simulink model "Es4_simulink"  (R2025b)
settings: Solver=VariableStepAuto  StartTime=0.0  StopTime=10.0  RelTol=1e-3
undefined symbols (not defined in the file): const_expr1, const_expr2, ramp_gain, step_gain
libraries: simulink x1
settings Model: Creator=fsisa  LastModifiedBy=fsisa

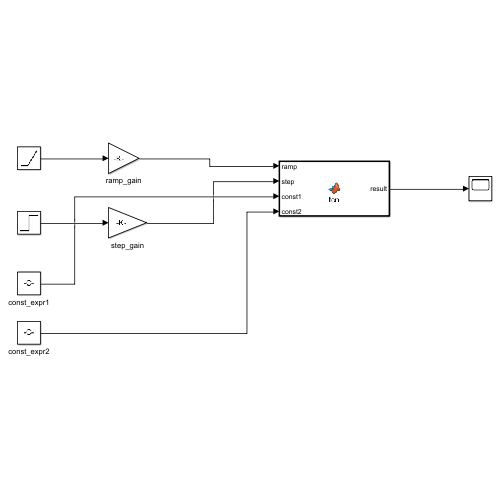
[thumbnail: Simulink's stored preview of the top-level diagram]
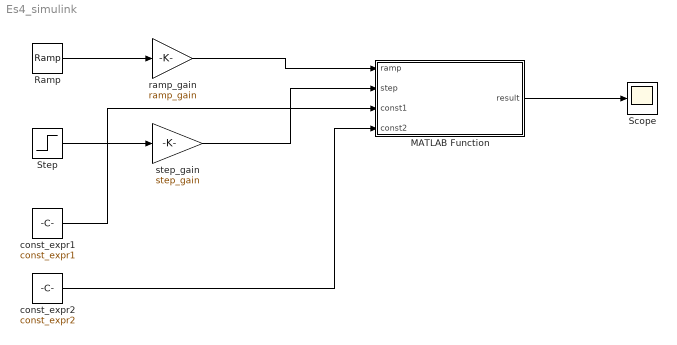
== system Es4_simulink ==
  MATLAB Function : MATLAB Function  TreatAsAtomicUnit=on
  Ramp : simulink/Sources/Ramp  slope=2  start=0  InitialOutput=0
  Scope : Scope
      settings: ActiveDisplayYMinimum=-6.7999999999999243  ActiveDisplayYMaximum=39.199999999999996
  Step : Step  Time=2  SampleTime=0
  const_expr1 : Constant  Value=const_expr1
  const_expr2 : Constant  Value=const_expr2
  ramp_gain : Gain  Gain=ramp_gain
  step_gain : Gain  Gain=step_gain
  wires:
  Ramp/1 -> ramp_gain/1
  Step/1 -> step_gain/1
  step_gain/1 -> MATLAB Function/2(step)
  ramp_gain/1 -> MATLAB Function/1(ramp)
  const_expr1/1 -> MATLAB Function/3(const1)
  const_expr2/1 -> MATLAB Function/4(const2)
  MATLAB Function/1(result) -> Scope/1

== matlab function Es4_simulink/MATLAB Function ==
  data: ramp input; step input; result output; const1 input; const2 input
function result = fcn(ramp, step, const1, const2)
    result = ramp/const1 - step*const2;
